simulink model "GripperBench"  (R2026b)
settings: Solver=daessc  StopTime=1  RelTol=1e-4
values from neighbouring files (symbols this model uses):
  P = struct('finger', fi, 'gas', ga, 'obj', o, 'bench', b)    [gripperBenchParams.m]
  X = [0 0 -1]    [gripperBenchParams.m]
  Y = -er    [gripperBenchParams.m]
  Z = cross(X, Y)    [gripperBenchParams.m]
libraries: sm_lib x44, nesl_utility x37
settings Model: Creator=amavromm  LastModifiedBy=amavromm
settings SimscapeCC: SimscapeNominalValues="[{\"value\":\"1\",\"unit\":\"A\"},{\"value\":\"1\",\"unit\":\"bar\"},{\"value\":\"1\",\"unit\":\"cm^2\"},{\"value\":\"1\",\"unit\":\"cm^3/s\"},{\"value\":\"1\",\"unit\":\"kJ/kg\"},{\"value\":\"1\",\"unit\":\"kW\"},{\"value\":\"1\",\"unit\":\"l\"},{\"value\":\"1\",\"unit\":\"N\"},{\"value\":\"1\",\"unit\":\"N*m\"},{\"value\":\"1\",\"unit\":\"V\"},{\"value\":\"0.001\",\"unit\":\"Wb\"}]"  SimscapeUseEnergyAccounting=off

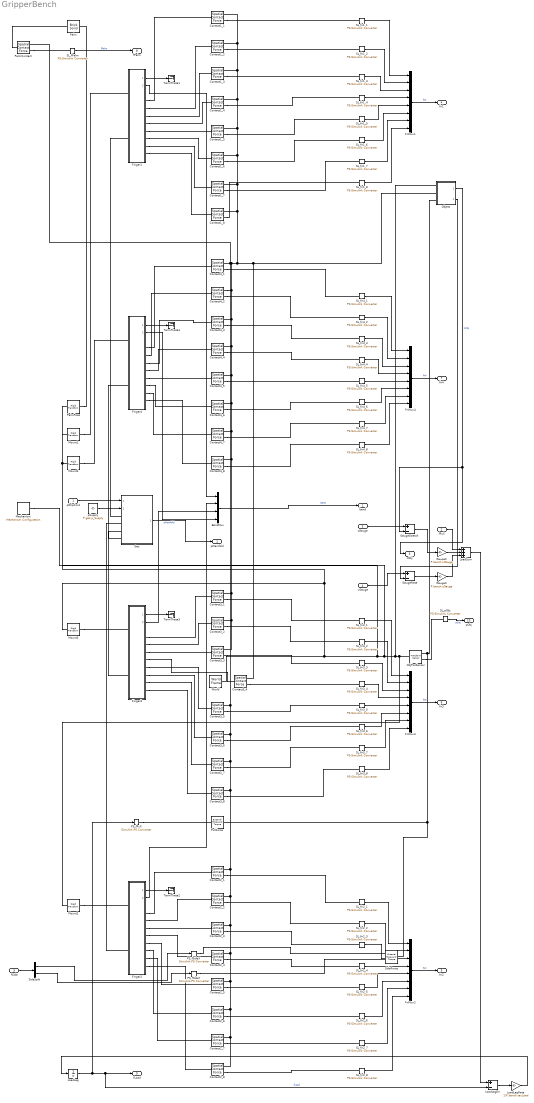
== system GripperBench ==
  pGripCmd : Inport
  fPull : Inport  Port=2
  zGauge : Inport  Port=3
  vGauge : Inport  Port=4
  fSide : Inport  Port=5  PortDimensions=2
  BendMux : Mux
  Contact1_{1..8} (8 alike) : sm_lib/Forces and Torques/Spatial Contact Force  SenseSeparationDistance=off  NormalForceType=SmoothSpringDamper  NormalStiffness=P.obj.k_Contact  NormalStiffnessUnits=N/m  NormalDamping=P.obj.c_Contact  NormalDampingUnits=N/(m/s)  NormalTransitionRegionWidth=P.bench.wContact  NormalTransitionRegionWidthUnits=m  FrictionType=SmoothStickSlip  CoefficientOfStaticFriction=P.obj.mu_s  CoefficientOfDynamicFriction=P.obj.mu_d  FrictionalCriticalVelocity=P.bench.vCrit  FrictionalCriticalVelocityUnits=m/s  SenseContactSignal=off  SensePenetrationDepth=off  SenseNormalVelocity=off  SenseTangentialVelocity=off  SensingForceTorqueDirection=BaseOnFollower  SensingForceTorqueResolutionFrame=ContactFrame  SenseNormalForce=off  SenseNormalForceMagnitude=on  SenseNormalTorque=off  SenseFrictionalForce=off  SenseFrictionalForceMagnitude=off  SenseFrictionalTorque=off  SenseTotalForce=off  SenseTotalTorque=off  SenseContactBaseRotation=off  SenseContactBaseTranslation=off  SenseContactFollowerRotation=off  SenseContactFollowerTranslation=off  ZeroCrossDetectContactStartAndEnd=off
  Contact2_{1..8} (8 alike) : sm_lib/Forces and Torques/Spatial Contact Force  SenseSeparationDistance=off  NormalForceType=SmoothSpringDamper  NormalStiffness=P.obj.k_Contact  NormalStiffnessUnits=N/m  NormalDamping=P.obj.c_Contact  NormalDampingUnits=N/(m/s)  NormalTransitionRegionWidth=P.bench.wContact  NormalTransitionRegionWidthUnits=m  FrictionType=SmoothStickSlip  CoefficientOfStaticFriction=P.obj.mu_s  CoefficientOfDynamicFriction=P.obj.mu_d  FrictionalCriticalVelocity=P.bench.vCrit  FrictionalCriticalVelocityUnits=m/s  SenseContactSignal=off  SensePenetrationDepth=off  SenseNormalVelocity=off  SenseTangentialVelocity=off  SensingForceTorqueDirection=BaseOnFollower  SensingForceTorqueResolutionFrame=ContactFrame  SenseNormalForce=off  SenseNormalForceMagnitude=on  SenseNormalTorque=off  SenseFrictionalForce=off  SenseFrictionalForceMagnitude=off  SenseFrictionalTorque=off  SenseTotalForce=off  SenseTotalTorque=off  SenseContactBaseRotation=off  SenseContactBaseTranslation=off  SenseContactFollowerRotation=off  SenseContactFollowerTranslation=off  ZeroCrossDetectContactStartAndEnd=off
  Contact3_{1..8} (8 alike) : sm_lib/Forces and Torques/Spatial Contact Force  SenseSeparationDistance=off  NormalForceType=SmoothSpringDamper  NormalStiffness=P.obj.k_Contact  NormalStiffnessUnits=N/m  NormalDamping=P.obj.c_Contact  NormalDampingUnits=N/(m/s)  NormalTransitionRegionWidth=P.bench.wContact  NormalTransitionRegionWidthUnits=m  FrictionType=SmoothStickSlip  CoefficientOfStaticFriction=P.obj.mu_s  CoefficientOfDynamicFriction=P.obj.mu_d  FrictionalCriticalVelocity=P.bench.vCrit  FrictionalCriticalVelocityUnits=m/s  SenseContactSignal=off  SensePenetrationDepth=off  SenseNormalVelocity=off  SenseTangentialVelocity=off  SensingForceTorqueDirection=BaseOnFollower  SensingForceTorqueResolutionFrame=ContactFrame  SenseNormalForce=off  SenseNormalForceMagnitude=on  SenseNormalTorque=off  SenseFrictionalForce=off  SenseFrictionalForceMagnitude=off  SenseFrictionalTorque=off  SenseTotalForce=off  SenseTotalTorque=off  SenseContactBaseRotation=off  SenseContactBaseTranslation=off  SenseContactFollowerRotation=off  SenseContactFollowerTranslation=off  ZeroCrossDetectContactStartAndEnd=off
  Contact4_{1..8} (8 alike) : sm_lib/Forces and Torques/Spatial Contact Force  SenseSeparationDistance=off  NormalForceType=SmoothSpringDamper  NormalStiffness=P.obj.k_Contact  NormalStiffnessUnits=N/m  NormalDamping=P.obj.c_Contact  NormalDampingUnits=N/(m/s)  NormalTransitionRegionWidth=P.bench.wContact  NormalTransitionRegionWidthUnits=m  FrictionType=SmoothStickSlip  CoefficientOfStaticFriction=P.obj.mu_s  CoefficientOfDynamicFriction=P.obj.mu_d  FrictionalCriticalVelocity=P.bench.vCrit  FrictionalCriticalVelocityUnits=m/s  SenseContactSignal=off  SensePenetrationDepth=off  SenseNormalVelocity=off  SenseTangentialVelocity=off  SensingForceTorqueDirection=BaseOnFollower  SensingForceTorqueResolutionFrame=ContactFrame  SenseNormalForce=off  SenseNormalForceMagnitude=on  SenseNormalTorque=off  SenseFrictionalForce=off  SenseFrictionalForceMagnitude=off  SenseFrictionalTorque=off  SenseTotalForce=off  SenseTotalTorque=off  SenseContactBaseRotation=off  SenseContactBaseTranslation=off  SenseContactFollowerRotation=off  SenseContactFollowerTranslation=off  ZeroCrossDetectContactStartAndEnd=off
  Finger{1..4} (4 alike) : Subsystem  ReferencedSubsystem=SoftFinger
  FnMux{1..4} (4 alike) : Mux  Inputs=8
  Gas : Subsystem  ReferencedSubsystem=GripperGas
  GaugeC : Gain  Gain=P.bench.cGauge
  GaugeK : Gain  Gain=P.bench.kGauge
  GaugeRate : Sum  Inputs=+-
  GaugeStretch : Sum  Inputs=+-
  LoadLag : Integrator
  LoadLagErr : Sum  Inputs=+-
  LoadLagRate : Gain  Gain=1/P.bench.tauLoad
  LoadSum : Sum  Inputs=+++
  Mechanism : sm_lib/Utilities/Mechanism Configuration  UniformGravity=Constant  GravityVector=P.bench.gravity  GravityVectorUnits=m/s^2  LinearizationDelta=0.001  JointModeTransitionNonlinearIterations=2
  Mount1 : sm_lib/Frames and Transforms/Rigid Transform  RotationMethod=RotationMatrix  FollAlignAxisA=+X  BaseAlignAxisA=+Y  FollAlignAxisB=+Y  BaseAlignAxisB=+Z  RotationStandardAxis=+Z  RotationAngle=0  RotationAngleUnits=deg  RotationArbitraryAxis=[0 0 1]  RotationSequenceAxes=FollowerAxes  RotationSequence=XYX  RotationSequenceAngles=[0 0 0]  RotationSequenceAnglesUnits=deg  RotationMatrix=P.bench.mountR(:,:,1)  Quaternion=[1 0 0 0]  TranslationMethod=Cartesian  TranslationCartesianOffset=P.bench.mountT(1,:)  TranslationCartesianOffsetUnits=m  TranslationStandardAxis=+Z  TranslationStandardOffset=0  TranslationStandardOffsetUnits=m  TranslationROffset=0  TranslationROffsetUnits=m  TranslationThetaOffset=0  TranslationThetaOffsetUnits=deg  TranslationZOffset=0  TranslationZOffsetUnits=m
  Mount2 : sm_lib/Frames and Transforms/Rigid Transform  RotationMethod=RotationMatrix  FollAlignAxisA=+X  BaseAlignAxisA=+Y  FollAlignAxisB=+Y  BaseAlignAxisB=+Z  RotationStandardAxis=+Z  RotationAngle=0  RotationAngleUnits=deg  RotationArbitraryAxis=[0 0 1]  RotationSequenceAxes=FollowerAxes  RotationSequence=XYX  RotationSequenceAngles=[0 0 0]  RotationSequenceAnglesUnits=deg  RotationMatrix=P.bench.mountR(:,:,2)  Quaternion=[1 0 0 0]  TranslationMethod=Cartesian  TranslationCartesianOffset=P.bench.mountT(2,:)  TranslationCartesianOffsetUnits=m  TranslationStandardAxis=+Z  TranslationStandardOffset=0  TranslationStandardOffsetUnits=m  TranslationROffset=0  TranslationROffsetUnits=m  TranslationThetaOffset=0  TranslationThetaOffsetUnits=deg  TranslationZOffset=0  TranslationZOffsetUnits=m
  Mount3 : sm_lib/Frames and Transforms/Rigid Transform  RotationMethod=RotationMatrix  FollAlignAxisA=+X  BaseAlignAxisA=+Y  FollAlignAxisB=+Y  BaseAlignAxisB=+Z  RotationStandardAxis=+Z  RotationAngle=0  RotationAngleUnits=deg  RotationArbitraryAxis=[0 0 1]  RotationSequenceAxes=FollowerAxes  RotationSequence=XYX  RotationSequenceAngles=[0 0 0]  RotationSequenceAnglesUnits=deg  RotationMatrix=P.bench.mountR(:,:,3)  Quaternion=[1 0 0 0]  TranslationMethod=Cartesian  TranslationCartesianOffset=P.bench.mountT(3,:)  TranslationCartesianOffsetUnits=m  TranslationStandardAxis=+Z  TranslationStandardOffset=0  TranslationStandardOffsetUnits=m  TranslationROffset=0  TranslationROffsetUnits=m  TranslationThetaOffset=0  TranslationThetaOffsetUnits=deg  TranslationZOffset=0  TranslationZOffsetUnits=m
  Mount4 : sm_lib/Frames and Transforms/Rigid Transform  RotationMethod=RotationMatrix  FollAlignAxisA=+X  BaseAlignAxisA=+Y  FollAlignAxisB=+Y  BaseAlignAxisB=+Z  RotationStandardAxis=+Z  RotationAngle=0  RotationAngleUnits=deg  RotationArbitraryAxis=[0 0 1]  RotationSequenceAxes=FollowerAxes  RotationSequence=XYX  RotationSequenceAngles=[0 0 0]  RotationSequenceAnglesUnits=deg  RotationMatrix=P.bench.mountR(:,:,4)  Quaternion=[1 0 0 0]  TranslationMethod=Cartesian  TranslationCartesianOffset=P.bench.mountT(4,:)  TranslationCartesianOffsetUnits=m  TranslationStandardAxis=+Z  TranslationStandardOffset=0  TranslationStandardOffsetUnits=m  TranslationROffset=0  TranslationROffsetUnits=m  TranslationThetaOffset=0  TranslationThetaOffsetUnits=deg  TranslationZOffset=0  TranslationZOffsetUnits=m
  ObjPosSensor : sm_lib/Frames and Transforms/Transform Sensor  ObservationFrame=World  ExpressedInFrame=World  RotationSequence=XYX  SenseAngle=off  SenseAxis=off  SenseQ=off  SenseR=off  SenseRotationSequence=off  SenseOmegaX=off  SenseOmegaY=off  SenseOmegaZ=off  SenseOmega=off  SenseQDot=off  SenseRDot=off  SenseRotationSequenceDot=off  SenseAlphaX=off  SenseAlphaY=off  SenseAlphaZ=off  SenseAlpha=off  SenseQDDot=off  SenseRDDot=off  SenseX=off  SenseY=off  SenseZ=off  SenseXYZ=on  SenseRad=off  SenseAzim=off  SenseDist=off  SenseInc=off  SenseXDot=off  SenseYDot=off  SenseZDot=off  SenseXYZDot=off  SenseRadDot=off  SenseAzimDot=off  SenseDistDot=off  SenseIncDot=off  SenseXDDot=off  SenseYDDot=off  SenseZDDot=off  SenseXYZDDot=off  SenseRadDDot=off  SenseAzimDDot=off  SenseDistDDot=off  SenseIncDDot=off
  Object : Subsystem  ReferencedSubsystem=ObjectBody
  PS_fPull : nesl_utility/Simulink-PS Converter  PhysicalDomain=network_engine_domain  SubClassName=ps_input  LeftPortType=input  RightPortType=output  PseudoPeriodic=off  Frequencies=[]  NoiseDistribution=none  NoiseParameters=[]  Unit=N  AffineConversion=off  FilteringAndDerivatives=provide  SimscapeFilterOrder=1  InputFilterTimeConstant=0.001  UdotUserProvided=0
  PS_fSideX : nesl_utility/Simulink-PS Converter  PhysicalDomain=network_engine_domain  SubClassName=ps_input  LeftPortType=input  RightPortType=output  PseudoPeriodic=off  Frequencies=[]  NoiseDistribution=none  NoiseParameters=[]  Unit=N  AffineConversion=off  FilteringAndDerivatives=provide  SimscapeFilterOrder=1  InputFilterTimeConstant=0.001  UdotUserProvided=0
  PS_fSideY : nesl_utility/Simulink-PS Converter  PhysicalDomain=network_engine_domain  SubClassName=ps_input  LeftPortType=input  RightPortType=output  PseudoPeriodic=off  Frequencies=[]  NoiseDistribution=none  NoiseParameters=[]  Unit=N  AffineConversion=off  FilteringAndDerivatives=provide  SimscapeFilterOrder=1  InputFilterTimeConstant=0.001  UdotUserProvided=0
  Palm : sm_lib/Body Elements/Brick Solid  BrickDimensions=[P.bench.wPalm P.bench.wPalm P.bench.tPalm]  BrickDimensionsUnits=m  ExportEntireGeometry=on  InertiaType=CalculateFromGeometry  BasedOnType=Density  Density=1000  DensityUnits=kg/m^3  Mass=1  MassUnits=kg  CenterOfMass=[0 0 0]  CenterOfMassUnits=m  MomentsOfInertia=[1 1 1]  MomentsOfInertiaUnits=kg*m^2  ProductsOfInertia=[0 0 0]  ProductsOfInertiaUnits=kg*m^2  GraphicType=FromGeometry  MarkerShape=Sphere  MarkerSize=10  GraphicVisPropType=SimpleVisualProperties  GraphicDiffuseColor=[0.7 0.7 0.75]  GraphicOpacity=1  GraphicSpecularColor=[0.5 0.5 0.5 1.0]  GraphicAmbientColor=[0.15 0.15 0.15 1.0]  GraphicEmissiveColor=[0.0 0.0 0.0 1.0]  GraphicShininess=75  DoExposeReferenceFrame=on  SerializedFrames=<Frames/>
  PalmContact : sm_lib/Forces and Torques/Spatial Contact Force  SenseSeparationDistance=off  NormalForceType=SmoothSpringDamper  NormalStiffness=P.obj.k_Table  NormalStiffnessUnits=N/m  NormalDamping=P.obj.c_Table  NormalDampingUnits=N/(m/s)  NormalTransitionRegionWidth=P.bench.wContact  NormalTransitionRegionWidthUnits=m  FrictionType=SmoothStickSlip  CoefficientOfStaticFriction=P.obj.mu_s  CoefficientOfDynamicFriction=P.obj.mu_d  FrictionalCriticalVelocity=P.bench.vCrit  FrictionalCriticalVelocityUnits=m/s  SenseContactSignal=off  SensePenetrationDepth=off  SenseNormalVelocity=off  SenseTangentialVelocity=off  SensingForceTorqueDirection=BaseOnFollower  SensingForceTorqueResolutionFrame=ContactFrame  SenseNormalForce=off  SenseNormalForceMagnitude=on  SenseNormalTorque=off  SenseFrictionalForce=off  SenseFrictionalForceMagnitude=off  SenseFrictionalTorque=off  SenseTotalForce=off  SenseTotalTorque=off  SenseContactBaseRotation=off  SenseContactBaseTranslation=off  SenseContactFollowerRotation=off  SenseContactFollowerTranslation=off  ZeroCrossDetectContactStartAndEnd=off
  PalmPose : sm_lib/Frames and Transforms/Rigid Transform  RotationMethod=None  FollAlignAxisA=+X  BaseAlignAxisA=+Y  FollAlignAxisB=+Y  BaseAlignAxisB=+Z  RotationStandardAxis=+Z  RotationAngle=0  RotationAngleUnits=deg  RotationArbitraryAxis=[0 0 1]  RotationSequenceAxes=FollowerAxes  RotationSequence=XYX  RotationSequenceAngles=[0 0 0]  RotationSequenceAnglesUnits=deg  RotationMatrix=[1 0 0;0 1 0;0 0 1]  Quaternion=[1 0 0 0]  TranslationMethod=Cartesian  TranslationCartesianOffset=[0 0 P.bench.tPalm/2]  TranslationCartesianOffsetUnits=m  TranslationStandardAxis=+Z  TranslationStandardOffset=0  TranslationStandardOffsetUnits=m  TranslationROffset=0  TranslationROffsetUnits=m  TranslationThetaOffset=0  TranslationThetaOffsetUnits=deg  TranslationZOffset=0  TranslationZOffsetUnits=m
  PullForce : sm_lib/Forces and Torques/External Force and Torque  EnableForceX=off  EnableForceY=off  EnableForceZ=on  EnableForce=off  ForceResolutionFrame=World  EnableTorqueX=off  EnableTorqueY=off  EnableTorqueZ=off  EnableTorque=off  TorqueResolutionFrame=AttachedFrame
  SL_fPalm : nesl_utility/PS-Simulink Converter  PhysicalDomain=network_engine_domain  SubClassName=ps_output  LeftPortType=input  RightPortType=output  PseudoPeriodic=off  Frequencies=[]  VectorFormat=inherit  Unit=N  AffineConversion=off
  SL_fn1_{1..8} (8 alike) : nesl_utility/PS-Simulink Converter  PhysicalDomain=network_engine_domain  SubClassName=ps_output  LeftPortType=input  RightPortType=output  PseudoPeriodic=off  Frequencies=[]  VectorFormat=inherit  Unit=N  AffineConversion=off
  SL_fn2_{1..8} (8 alike) : nesl_utility/PS-Simulink Converter  PhysicalDomain=network_engine_domain  SubClassName=ps_output  LeftPortType=input  RightPortType=output  PseudoPeriodic=off  Frequencies=[]  VectorFormat=inherit  Unit=N  AffineConversion=off
  SL_fn3_{1..8} (8 alike) : nesl_utility/PS-Simulink Converter  PhysicalDomain=network_engine_domain  SubClassName=ps_output  LeftPortType=input  RightPortType=output  PseudoPeriodic=off  Frequencies=[]  VectorFormat=inherit  Unit=N  AffineConversion=off
  SL_fn4_{1..8} (8 alike) : nesl_utility/PS-Simulink Converter  PhysicalDomain=network_engine_domain  SubClassName=ps_output  LeftPortType=input  RightPortType=output  PseudoPeriodic=off  Frequencies=[]  VectorFormat=inherit  Unit=N  AffineConversion=off
  SL_pObj : nesl_utility/PS-Simulink Converter  PhysicalDomain=network_engine_domain  SubClassName=ps_output  LeftPortType=input  RightPortType=output  PseudoPeriodic=off  Frequencies=[]  VectorFormat=inherit  Unit=m  AffineConversion=off
  SideForce : sm_lib/Forces and Torques/External Force and Torque  EnableForceX=on  EnableForceY=on  EnableForceZ=off  EnableForce=off  ForceResolutionFrame=World  EnableTorqueX=off  EnableTorqueY=off  EnableTorqueZ=off  EnableTorque=off  TorqueResolutionFrame=AttachedFrame
  SideSplit : Demux  Outputs=2
  TermTheta{1..4} (4 alike) : Terminator
  World : sm_lib/Frames and Transforms/World Frame
  pSupply : Constant  Value=P.gas.p_Supply
  bend : Outport
  pManifold : Outport  Port=2
  zObj : Outport  Port=3
  fn1 : Outport  Port=4
  fn2 : Outport  Port=5
  fn3 : Outport  Port=6
  fn4 : Outport  Port=7
  fPalm : Outport  Port=8
  fLoad : Outport  Port=9
  pObj : Outport  Port=10
  wires:
  LoadLagRate/1 -> LoadLag/1
  LoadLagErr/1 -> LoadLagRate/1
  LoadLag/1 -> LoadLagErr/2, fLoad/1, PS_fPull/1  "fLoad"
  LoadSum/1 -> LoadLagErr/1
  GaugeC/1 -> LoadSum/3
  GaugeK/1 -> LoadSum/2
  GaugeRate/1 -> GaugeC/1
  vGauge/1 -> GaugeRate/1
  GaugeStretch/1 -> GaugeK/1
  zGauge/1 -> GaugeStretch/1
  FnMux3/1 -> fn3/1  "fn3"
  SL_fn3_8/1 -> FnMux3/8
  SL_fn3_7/1 -> FnMux3/7
  SL_fn3_6/1 -> FnMux3/6
  SL_fn3_5/1 -> FnMux3/5
  SL_fn3_4/1 -> FnMux3/4
  SL_fn3_3/1 -> FnMux3/3
  SL_fn3_2/1 -> FnMux3/2
  SL_fn3_1/1 -> FnMux3/1
  Finger4/1 -> TermTheta4/1
  Finger3/1 -> TermTheta3/1
  Finger2/1 -> TermTheta2/1
  Finger1/1 -> TermTheta1/1
  BendMux/1 -> bend/1  "bend"
  Finger4/2 -> BendMux/4
  Finger3/2 -> BendMux/3
  Finger2/2 -> BendMux/2
  Finger1/2 -> BendMux/1
  fPull/1 -> LoadSum/1
  Gas/1 -> pManifold/1  "pManifold"
  pSupply/1 -> Gas/2
  pGripCmd/1 -> Gas/1
  SL_fn1_1/1 -> FnMux1/1
  SL_fn1_2/1 -> FnMux1/2
  SL_fn1_3/1 -> FnMux1/3
  SL_fn1_4/1 -> FnMux1/4
  SL_fn1_5/1 -> FnMux1/5
  SL_fn1_6/1 -> FnMux1/6
  SL_fn1_7/1 -> FnMux1/7
  SL_fn1_8/1 -> FnMux1/8
  FnMux1/1 -> fn1/1  "fn1"
  SL_fn2_1/1 -> FnMux2/1
  SL_fn2_2/1 -> FnMux2/2
  SL_fn2_3/1 -> FnMux2/3
  SL_fn2_4/1 -> FnMux2/4
  SL_fn2_5/1 -> FnMux2/5
  SL_fn2_6/1 -> FnMux2/6
  SL_fn2_7/1 -> FnMux2/7
  SL_fn2_8/1 -> FnMux2/8
  FnMux2/1 -> fn2/1  "fn2"
  SL_fn4_1/1 -> FnMux4/1
  SL_fn4_2/1 -> FnMux4/2
  SL_fn4_3/1 -> FnMux4/3
  SL_fn4_4/1 -> FnMux4/4
  SL_fn4_5/1 -> FnMux4/5
  SL_fn4_6/1 -> FnMux4/6
  SL_fn4_7/1 -> FnMux4/7
  SL_fn4_8/1 -> FnMux4/8
  FnMux4/1 -> fn4/1  "fn4"
  SL_fPalm/1 -> fPalm/1  "fPalm"
  SideSplit/2 -> PS_fSideY/1
  SideSplit/1 -> PS_fSideX/1
  fSide/1 -> SideSplit/1
  SL_pObj/1 -> pObj/1  "pObj"
  Object/2 -> GaugeRate/2
  Object/1 -> zObj/1, GaugeStretch/2  "zObj"
  connections:
  Contact3_8/RConn2 -- SL_fn3_8/LConn1
  Contact3_7/RConn2 -- SL_fn3_7/LConn1
  Contact3_6/RConn2 -- SL_fn3_6/LConn1
  Contact3_5/RConn2 -- SL_fn3_5/LConn1
  Contact3_3/RConn2 -- SL_fn3_3/LConn1
  Contact3_2/RConn2 -- SL_fn3_2/LConn1
  Contact3_1/RConn2 -- SL_fn3_1/LConn1
  Finger3/RConn9 -- Contact3_8/LConn1
  Finger3/RConn8 -- Contact3_7/LConn1
  Finger3/RConn7 -- Contact3_6/LConn1
  Finger3/RConn6 -- Contact3_5/LConn1
  Finger3/RConn4 -- Contact3_3/LConn1
  Finger3/RConn3 -- Contact3_2/LConn1
  Finger3/RConn2 -- Contact3_1/LConn1
  Contact1_8/RConn2 -- SL_fn1_8/LConn1
  Contact1_7/RConn2 -- SL_fn1_7/LConn1
  Contact1_6/RConn2 -- SL_fn1_6/LConn1
  Contact1_5/RConn2 -- SL_fn1_5/LConn1
  Contact1_4/RConn2 -- SL_fn1_4/LConn1
  Contact1_3/RConn2 -- SL_fn1_3/LConn1
  Contact1_2/RConn2 -- SL_fn1_2/LConn1
  Contact1_1/RConn2 -- SL_fn1_1/LConn1
  PS_fPull/RConn1 -- PullForce/LConn1
  Gas/LConn4 -- Finger4/LConn2
  Gas/LConn3 -- Finger3/LConn2
  Gas/LConn2 -- Finger2/LConn2
  Gas/LConn1 -- Finger1/LConn2
  Mount4/RConn1 -- Finger4/LConn1
  Mount3/RConn1 -- Finger3/LConn1
  Mount2/RConn1 -- Finger2/LConn1
  Mount1/RConn1 -- Finger1/LConn1
  Finger1/RConn2 -- Contact1_1/LConn1
  Finger1/RConn3 -- Contact1_2/LConn1
  Finger1/RConn4 -- Contact1_3/LConn1
  Finger1/RConn5 -- Contact1_4/LConn1
  Finger1/RConn6 -- Contact1_5/LConn1
  Finger1/RConn7 -- Contact1_6/LConn1
  Finger1/RConn8 -- Contact1_7/LConn1
  Finger1/RConn9 -- Contact1_8/LConn1
  Finger2/RConn2 -- Contact2_1/LConn1
  Finger2/RConn3 -- Contact2_2/LConn1
  Finger2/RConn4 -- Contact2_3/LConn1
  Finger2/RConn5 -- Contact2_4/LConn1
  Finger2/RConn6 -- Contact2_5/LConn1
  Finger2/RConn7 -- Contact2_6/LConn1
  Finger2/RConn8 -- Contact2_7/LConn1
  Finger2/RConn9 -- Contact2_8/LConn1
  Contact2_1/RConn2 -- SL_fn2_1/LConn1
  Contact2_2/RConn2 -- SL_fn2_2/LConn1
  Contact2_3/RConn2 -- SL_fn2_3/LConn1
  Contact2_4/RConn2 -- SL_fn2_4/LConn1
  Contact2_5/RConn2 -- SL_fn2_5/LConn1
  Contact2_6/RConn2 -- SL_fn2_6/LConn1
  Contact2_7/RConn2 -- SL_fn2_7/LConn1
  Contact2_8/RConn2 -- SL_fn2_8/LConn1
  Finger4/RConn2 -- Contact4_1/LConn1
  Finger4/RConn3 -- Contact4_2/LConn1
  Finger4/RConn4 -- Contact4_3/LConn1
  Finger4/RConn5 -- Contact4_4/LConn1
  Finger4/RConn6 -- Contact4_5/LConn1
  Finger4/RConn7 -- Contact4_6/LConn1
  Finger4/RConn8 -- Contact4_7/LConn1
  Finger4/RConn9 -- Contact4_8/LConn1
  Contact4_1/RConn2 -- SL_fn4_1/LConn1
  Contact4_2/RConn2 -- SL_fn4_2/LConn1
  Contact4_3/RConn2 -- SL_fn4_3/LConn1
  Contact4_4/RConn2 -- SL_fn4_4/LConn1
  Contact4_5/RConn2 -- SL_fn4_5/LConn1
  Contact4_6/RConn2 -- SL_fn4_6/LConn1
  Contact4_7/RConn2 -- SL_fn4_7/LConn1
  Contact4_8/RConn2 -- SL_fn4_8/LConn1
  PalmPose/RConn1 -- Palm/RConn1
  Palm/LConn1 -- PalmContact/LConn1
  PalmContact/RConn2 -- SL_fPalm/LConn1
  PS_fSideY/RConn1 -- SideForce/LConn2
  PS_fSideX/RConn1 -- SideForce/LConn1
  SideForce/RConn1 -- ObjPosSensor/RConn1 -- Object/LConn3 -- PullForce/RConn1
  Mechanism/RConn1 -- Mount1/LConn1 -- Mount4/LConn1 -- Mount3/LConn1 -- World/RConn1 -- PalmPose/LConn1 -- ObjPosSensor/LConn1 -- Mount2/LConn1 -- Object/LConn1
  Contact4_2/RConn1 -- Contact3_2/RConn1 -- Contact3_3/RConn1 -- Contact3_1/RConn1 -- Contact4_8/RConn1 -- Contact4_7/RConn1 -- Contact4_6/RConn1 -- Contact4_5/RConn1 -- Contact4_4/RConn1 -- Contact4_3/RConn1 -- Object/LConn2 -- Contact3_4/RConn1 -- Contact1_2/RConn1 -- Contact1_1/RConn1 -- Contact1_3/RConn1 -- Contact1_4/RConn1 -- Contact1_5/RConn1 -- Contact1_6/RConn1 -- Contact1_7/RConn1 -- Contact1_8/RConn1 -- Contact2_8/RConn1 -- Contact2_7/RConn1 -- Contact2_6/RConn1 -- Contact2_5/RConn1 -- Contact2_4/RConn1 -- Contact2_3/RConn1 -- Contact2_2/RConn1 -- Contact2_1/RConn1 -- Contact3_8/RConn1 -- Contact3_7/RConn1 -- Contact3_6/RConn1 -- Contact3_5/RConn1 -- Contact4_1/RConn1 -- PalmContact/RConn1
  ObjPosSensor/RConn2 -- SL_pObj/LConn1
  Finger3/RConn5 -- Contact3_4/LConn1
  Contact3_4/RConn2 -- SL_fn3_4/LConn1
